simulink model "Boost_Source_Open_Loop"  (R2024b)
settings: Solver=FixedStepAuto  StartTime=0.0  StopTime=10  MaxStep=1e-4  RelTol=1e-3
libraries: spsSeriesRLCBranchLib x3, spsCurrentMeasurementLib x2, spsDCVoltageSourceLib x1, spsDiodeLib x1, spsMosfetLib x1, spsPWMGeneratorDCDCLib x1, spsVoltageMeasurementLib x1, spspowerguiLib x1
settings Model: Creator=Parti  LastModifiedBy=Eng.Abd-Elrhman Saad

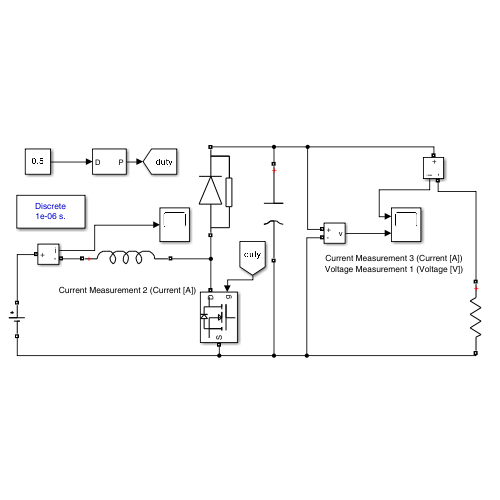
[thumbnail: Simulink's stored preview of the top-level diagram]
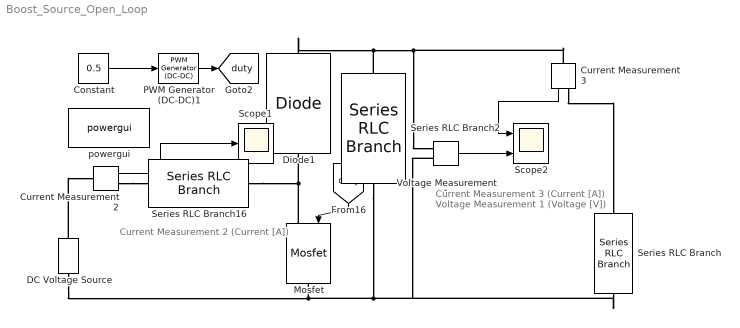
== system Boost_Source_Open_Loop ==
  note: Current Measurement 2 (Current [A])
  note: Current Measurement 3 (Current [A])
      | Voltage Measurement 1 (Voltage [V])
  Constant : Constant  Value=0.5
  Current Measurement2 : spsCurrentMeasurementLib/Current Measurement  PhasorSimulation=off  OutputType=Complex  PSBequivalent=0
  Current Measurement3 : spsCurrentMeasurementLib/Current Measurement  PhasorSimulation=off  OutputType=Complex  PSBequivalent=0
  DC Voltage Source : spsDCVoltageSourceLib/DC Voltage Source  Amplitude=12  Measurements=None
  Diode1 : spsDiodeLib/Diode  Ron=0.001  Lon=0  Vf=0.8  IC=0  UseSnubber=0  Rs=500  Cs=250e-9  Measurements=off
  Mosfet : spsMosfetLib/Mosfet  Ron=0.1  Lon=0  Rd=0.01  Vfd=0  IC=0  Rs=1e5  Cs=inf  Measurements=off
  PWM Generator (DC-DC)1 : spsPWMGeneratorDCDCLib/PWM Generator (DC-DC)  Fsw=10000  Ts=1e-6
  Scope1 : Scope
  Scope2 : Scope  NumInputPorts=2
  Series RLC Branch : spsSeriesRLCBranchLib/Series RLC Branch  LConnTagsString=__new0  RConnTagsString=__new0  BranchType=R  Resistance=220  Inductance=1e-3  SetiL0=off  InitialCurrent=0  Capacitance=1e-6  Setx0=off  InitialVoltage=0  Measurements=None
  Series RLC Branch16 : spsSeriesRLCBranchLib/Series RLC Branch  LConnTagsString=__new0  RConnTagsString=__new0  BranchType=L  Resistance=1  Inductance=2e-3  SetiL0=off  InitialCurrent=0  Capacitance=1000e-6  Setx0=on  InitialVoltage=100  Measurements=None
  Series RLC Branch2 : spsSeriesRLCBranchLib/Series RLC Branch  LConnTagsString=__new0  RConnTagsString=__new0  BranchType=C  Resistance=1  Inductance=1e-3  SetiL0=off  InitialCurrent=0  Capacitance=2e-3  Setx0=on  InitialVoltage=0  Measurements=None
  Voltage Measurement1 : spsVoltageMeasurementLib/Voltage Measurement  PhasorSimulation=off  OutputType=Complex  PSBequivalent=0
  powergui : spspowerguiLib/powergui  Priority=1  SimulationMode=Discrete  SampleTime=1e-6  frequency=60  Iterations=50  frequencyindice=0  Pbase=100e6  ErrMax=1e-4  UnitsV=kV  UnitsW=MW  buscounter=0  FunctionMessages=off  echomessages=off  EnableUseOfTLC=off  CurrentSourceSwitches=off  DisableSnubberDevices=off  DisableRonSwitches=off  DisableVfSwitches=off  DisplayEquations=off  AutomaticDiscreteSolvers=off  SolverType=Tustin/Backward Euler (TBE)  Interpol=off  ExternalGateDelay=off  methode=off  Ts=100  x0status=blocks  SPID=on  SwTol=0  HookPort=off  NonlinearTolerance=1e-4  nMaxIteration=100  ContinueOnMaxIteration=off  RestoreLinks=warning  ResistiveCurrentMeasurement=off  Frange=[0:2:500]  Ylog=off  Xlog=on  ShowGrid=off  save=off  variable=ZData  structure=0  ZoomFFT=off  StartTime=0.0  cycles=1  DisplayStyle=1  fundamental=60  FreqAxis=off  MaxFrequency=1000  frequencyindicesteady=1  RmsSteady=1  display=off
  tag scope: duty=global
  wires:
  [duty] -> Mosfet/1
  Current Measurement3/1 -> Scope2/1
  Constant/1 -> PWM Generator (DC-DC)1/1
  PWM Generator (DC-DC)1/1 -> [duty]
  Current Measurement2/1 -> Scope1/1
  Voltage Measurement1/1 -> Scope2/2
  connections:
  Series RLC Branch16/RConn1 -- Mosfet/LConn1 -- Diode1/LConn1
  Diode1/RConn1 -- Current Measurement3/LConn1 -- Voltage Measurement1/LConn1 -- Series RLC Branch2/LConn1
  Series RLC Branch2/RConn1 -- Series RLC Branch/RConn1 -- Voltage Measurement1/LConn2 -- DC Voltage Source/LConn1 -- Mosfet/RConn1
  DC Voltage Source/RConn1 -- Current Measurement2/LConn1
  Current Measurement2/RConn1 -- Series RLC Branch16/LConn1
  Current Measurement3/RConn1 -- Series RLC Branch/LConn1
